simulink model "task3_simulation"  (R2025b)
settings: Solver=FixedStepAuto  StartTime=0.0  StopTime=45.4159  RelTol=1e-3
undefined symbols (not defined in the file): d, DiscIntNeverNeededParam, is_real_robot, k_theta, k_x, k_y, q_init, r, Ts, X, Y
libraries: robotlib x6, sharedtransform x1
settings Model: Creator=dallaliber  LastModifiedBy=ilia
settings OptimizationCC: DefaultParameterBehavior=Inlined  EnhancedBackFolding=on  PassReuseOutputArgsAs=Individual arguments  ZeroExternalMemoryAtStartup=off  ZeroInternalMemoryAtStartup=off  MaxStackSize=64  OptimizeBlockOrder=speed  DifferentSizesBufferReuse=on  OptimizationCustomize=off  EfficientTunableParamExpr=on
settings DebuggingCC: ParameterTunabilityLossMsg=error
settings HardwareCC: ProdBitPerPointer=32.0  ProdBitPerSizeT=32.0  ProdBitPerPtrDiffT=32.0  ProdLargestAtomicFloat=None  ProdIntDivRoundTo=Undefined  ProdEndianess=Unspecified  ProdWordSize=32.0  ProdHWDeviceType=Generic->Unspecified (assume 32-bit Generic)
settings SFSimCC: MATLABDynamicMemAlloc=off
settings RTWCC: SystemTargetFile=ert.tlc  HardwareBoard=Robot Operating System (ROS)  TLCOptions="-aInlineSetEventsForThisBaseRateFcn=TLC_FALSE -aSuppressMultiTaskScheduler=TLC_FALSE  -aRateBasedStepFcn=0"  TemplateMakefile=ert_default_tmf  Toolchain=Catkin  TargetLang=C++  Description=Embedded Coder
settings CodeAppCC: ForceParamTrailComments=on  IgnoreCustomStorageClasses=off  OperatorAnnotations=on  SimulinkDataObjDesc=on  SFDataObjDesc=on  InsertBlockDesc=on
settings ERTTargetCC: DynamicArrayContainerType=coder::array

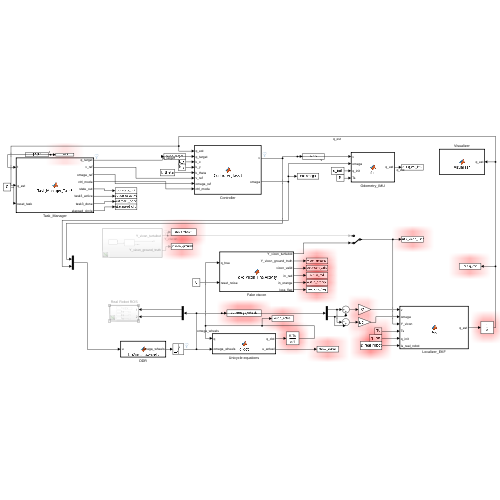
[thumbnail: Simulink's stored preview of the top-level diagram]
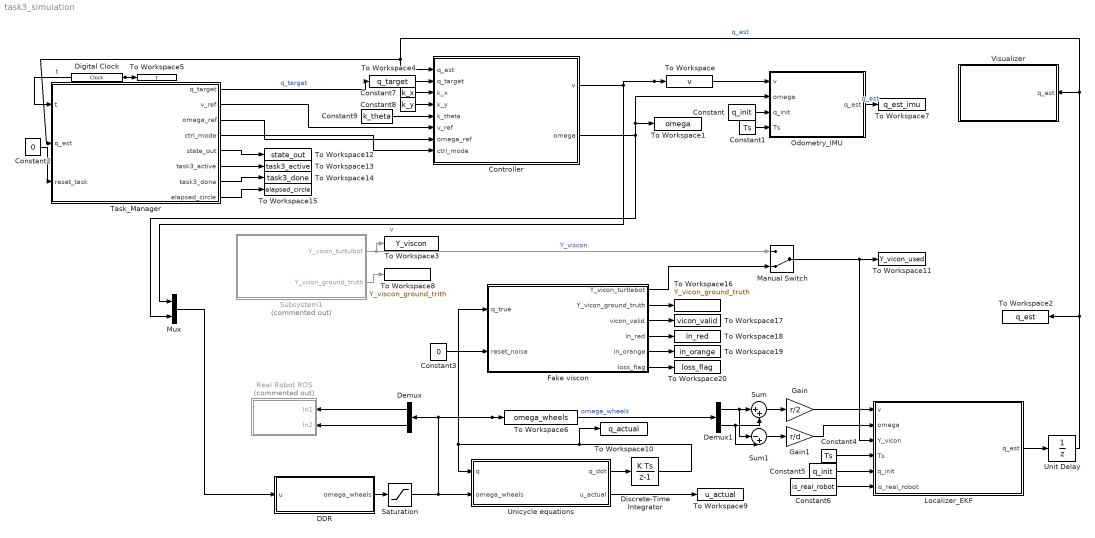
== system task3_simulation ==
  Constant : Constant  Value=q_init  SampleTime=Ts
  Constant1 : Constant  Value=Ts  SampleTime=Ts
  Constant2 : Constant  Value=0
  Constant3 : Constant  Value=0
  Constant4 : Constant  Value=Ts
  Constant5 : Constant  Value=q_init
  Constant6 : Constant  Value=is_real_robot
  Constant7 : Constant  Value=k_x  SampleTime=Ts
  Constant8 : Constant  Value=k_y  SampleTime=Ts
  Constant9 : Constant  Value=k_theta  SampleTime=Ts
  Controller : MATLAB Function  TreatAsAtomicUnit=on
  DDR : MATLAB Function  TreatAsAtomicUnit=on
  Demux : Demux  Outputs=2
  Demux1 : Demux  Outputs=2
  Digital Clock : DigitalClock  SampleTime=Ts
  Discrete-Time Integrator : DiscreteIntegrator  InitialCondition=q_init  SampleTime=Ts  ICPrevOutput=DiscIntNeverNeededParam  ICPrevScaledInput=DiscIntNeverNeededParam
  Fake viscon : MATLAB Function  TreatAsAtomicUnit=on
  Gain : Gain  Gain=r/2
  Gain1 : Gain  Gain=r/d
  Localizer_EKF : MATLAB Function  TreatAsAtomicUnit=on
  Manual Switch : ManualSwitch  CurrentSetting=0
  Mux : Mux  Inputs=2
  Odometry_IMU : MATLAB Function  TreatAsAtomicUnit=on
  Real Robot ROS : Subsystem  Commented=on
  Saturation : Saturate  UpperLimit=10  LowerLimit=-10
  Subsystem1 : Subsystem  Commented=on
  Sum : Sum  Inputs=|++
  Sum1 : Sum  Inputs=|-+
  Task_Manager : MATLAB Function  TreatAsAtomicUnit=on
  To Workspace : ToWorkspace  VariableName=v  SampleTime=Ts
  To Workspace1 : ToWorkspace  VariableName=omega  SampleTime=Ts
  To Workspace10 : ToWorkspace  VariableName=q_actual  SampleTime=Ts
  To Workspace11 : ToWorkspace  VariableName=Y_vicon_used  SampleTime=Ts
  To Workspace12 : ToWorkspace  VariableName=state_out  SampleTime=Ts
  To Workspace13 : ToWorkspace  VariableName=task3_active  SampleTime=Ts
  To Workspace14 : ToWorkspace  VariableName=task3_done  SampleTime=Ts
  To Workspace15 : ToWorkspace  VariableName=elapsed_circle  SampleTime=Ts
  To Workspace16 : ToWorkspace  VariableName=Y_vicon_ground_truth  SampleTime=Ts
  To Workspace17 : ToWorkspace  VariableName=vicon_valid  SampleTime=Ts
  To Workspace18 : ToWorkspace  VariableName=in_red  SampleTime=Ts
  To Workspace19 : ToWorkspace  VariableName=in_orange  SampleTime=Ts
  To Workspace2 : ToWorkspace  VariableName=q_est  SampleTime=Ts
  To Workspace20 : ToWorkspace  VariableName=loss_flag  SampleTime=Ts
  To Workspace3 : ToWorkspace  VariableName=Y_viscon  SampleTime=Ts
  To Workspace4 : ToWorkspace  VariableName=q_target  SampleTime=Ts
  To Workspace5 : ToWorkspace  VariableName=t  SampleTime=Ts
  To Workspace6 : ToWorkspace  VariableName=omega_wheels  SampleTime=Ts
  To Workspace7 : ToWorkspace  VariableName=q_est_imu  SampleTime=Ts
  To Workspace8 : ToWorkspace  VariableName=Y_viscon_ground_trith  SampleTime=Ts
  To Workspace9 : ToWorkspace  VariableName=u_actual  SampleTime=Ts
  Unicycle equations : MATLAB Function  TreatAsAtomicUnit=on
  Unit Delay : UnitDelay  InitialCondition=q_init  SampleTime=Ts  HasFrameUpgradeWarning=on
  Visualizer : MATLAB Function  TreatAsAtomicUnit=on
  wires:
  Controller/1(v) -> Odometry_IMU/1(v), To Workspace/1, Mux/1  "v"
  Constant/1 -> Odometry_IMU/3(q_init)
  Constant1/1 -> Odometry_IMU/4(Ts)
  Odometry_IMU/1(q_est) -> To Workspace7/1  "q_est"
  Saturation/1 -> Demux/1, To Workspace6/1, Demux1/1, Unicycle equations/2(omega_wheels)  "omega_wheels"
  DDR/1(omega_wheels) -> Saturation/1
  Demux/1 -> Real Robot ROS/1(In1)
  Mux/1 -> DDR/1(u)
  Digital Clock/1 -> To Workspace5/1, Task_Manager/1(t)  "t"
  Unit Delay/1 -> Controller/1(q_est), Task_Manager/2(q_est), Visualizer/1(q_est), To Workspace2/1  "q_est"
  Subsystem1/1(Y_vicon_turtulbot) -> To Workspace3/1, Manual Switch/1  "Y_viscon"
  Task_Manager/1(q_target) -> Controller/2(q_target), To Workspace4/1  "q_target"
  Constant7/1 -> Controller/3(k_x)
  Constant8/1 -> Controller/4(k_y)
  Subsystem1/2(Y_vicon_ground_truth) -> To Workspace8/1
  Constant9/1 -> Controller/5(k_theta)
  Controller/2(omega) -> To Workspace1/1, Odometry_IMU/2(omega), Mux/2
  Unicycle equations/1(q_dot) -> Discrete-Time Integrator/1
  Discrete-Time Integrator/1 -> To Workspace10/1, Unicycle equations/1(q), Fake viscon/1(q_true)
  Unicycle equations/2(u_actual) -> To Workspace9/1
  Fake viscon/1(Y_vicon_turtlebot) -> Manual Switch/2
  Constant4/1 -> Localizer_EKF/4(Ts)
  Constant6/1 -> Localizer_EKF/6(is_real_robot)
  Constant5/1 -> Localizer_EKF/5(q_init)
  Localizer_EKF/1(q_est) -> Unit Delay/1
  Demux/2 -> Real Robot ROS/2(In2)
  Demux1/1 -> Sum1/1, Sum/1
  Demux1/2 -> Sum/2, Sum1/2
  Sum/1 -> Gain/1
  Gain/1 -> Localizer_EKF/1(v)
  Sum1/1 -> Gain1/1
  Gain1/1 -> Localizer_EKF/2(omega)
  Manual Switch/1 -> To Workspace11/1, Localizer_EKF/3(Y_vicon)
  Constant2/1 -> Task_Manager/3(reset_task)
  Task_Manager/2(v_ref) -> Controller/6(v_ref)
  Constant3/1 -> Fake viscon/2(reset_noise)
  Fake viscon/2(Y_vicon_ground_truth) -> To Workspace16/1
  Fake viscon/3(vicon_valid) -> To Workspace17/1
  Fake viscon/4(in_red) -> To Workspace18/1
  Fake viscon/5(in_orange) -> To Workspace19/1
  Fake viscon/6(loss_flag) -> To Workspace20/1
  Task_Manager/3(omega_ref) -> Controller/7(omega_ref)
  Task_Manager/4(ctrl_mode) -> Controller/8(ctrl_mode)
  Task_Manager/5(state_out) -> To Workspace12/1
  Task_Manager/6(task3_active) -> To Workspace13/1
  Task_Manager/7(task3_done) -> To Workspace14/1
  Task_Manager/8(elapsed_circle) -> To Workspace15/1

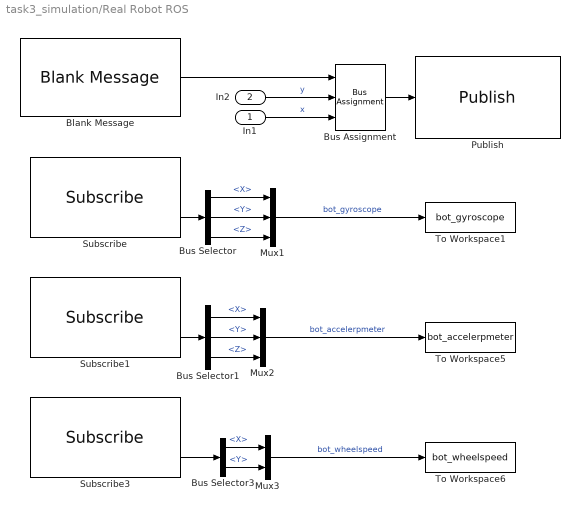
== system task3_simulation/Real Robot ROS ==
  In1 : Inport
  In2 : Inport  Port=2
  Blank Message : robotlib/Blank Message  messageClass=Message  entityType=geometry_msgs/Vector3  messageType=geometry_msgs/Vector3  SampleTime=0.04  legacyBusStruct=off
  Bus Assignment : BusAssignment  AssignedSignals=X,Y
  Bus Selector : BusSelector  OutputSignals=X,Y,Z
  Bus Selector1 : BusSelector  OutputSignals=X,Y,Z
  Bus Selector3 : BusSelector  OutputSignals=X,Y
  Mux1 : Mux  Inputs=3
  Mux2 : Mux  Inputs=3
  Mux3 : Mux  Inputs=2
  Publish : robotlib/Publish  topicSource=Select from ROS network  topic=/turtlebot_09/cmd_wheels  messageType=geometry_msgs/Vector3  legacyBusStruct=off  messageQueueLength=1
  Subscribe : robotlib/Subscribe  topicSource=Select from ROS network  topic=/turtlebot_09/gyroscope  messageType=geometry_msgs/Vector3  SampleTime=0.04  legacyBusStruct=off  messageQueueLength=1
  Subscribe1 : robotlib/Subscribe  topicSource=Select from ROS network  topic=/turtlebot_09/accelerometer  messageType=geometry_msgs/Vector3  SampleTime=0.04  legacyBusStruct=off  messageQueueLength=1
  Subscribe3 : robotlib/Subscribe  topicSource=Select from ROS network  topic=/turtlebot_09/wheelSpeeds  messageType=geometry_msgs/Vector3  SampleTime=0.04  legacyBusStruct=off  messageQueueLength=1
  To Workspace1 : ToWorkspace  VariableName=bot_gyroscope  SaveFormat=Timeseries  SampleTime=Ts
  To Workspace5 : ToWorkspace  VariableName=bot_accelerpmeter  SaveFormat=Timeseries  SampleTime=Ts
  To Workspace6 : ToWorkspace  VariableName=bot_wheelspeed  SaveFormat=Timeseries  SampleTime=Ts
  wires:
  Subscribe1/2 -> Bus Selector1/1
  Bus Selector1/1 -> Mux2/1  "<X>"
  Mux2/1 -> To Workspace5/1  "bot_accelerpmeter"
  Bus Assignment/1 -> Publish/1
  Subscribe/2 -> Bus Selector/1
  Bus Selector/2 -> Mux1/2  "<Y>"
  Bus Selector/1 -> Mux1/1  "<X>"
  Bus Selector3/1 -> Mux3/1  "<X>"
  Bus Selector3/2 -> Mux3/2  "<Y>"
  Bus Selector1/3 -> Mux2/3  "<Z>"
  Bus Selector1/2 -> Mux2/2  "<Y>"
  Mux3/1 -> To Workspace6/1  "bot_wheelspeed"
  Mux1/1 -> To Workspace1/1  "bot_gyroscope"
  Subscribe3/2 -> Bus Selector3/1
  Blank Message/1 -> Bus Assignment/1
  Bus Selector/3 -> Mux1/3  "<Z>"
  In1/1 -> Bus Assignment/3  "x"
  In2/1 -> Bus Assignment/2  "y"

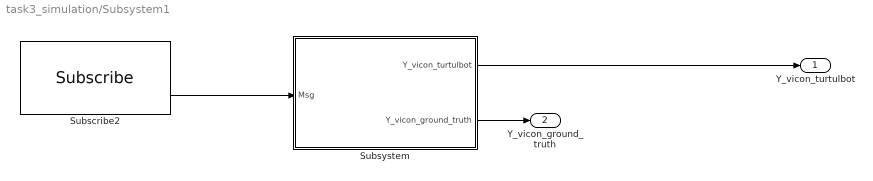
== system task3_simulation/Subsystem1 ==
  Subscribe2 : robotlib/Subscribe  topicSource=Select from ROS network  topic=/turtlebot_09/odom  messageType=nav_msgs/Odometry  SampleTime=Ts  legacyBusStruct=off  messageQueueLength=1
      settings: LibrarySourceBlock=roslib/ROS/Subscribe
  Subsystem : Subsystem
  Y_vicon_turtulbot : Outport
  Y_vicon_ground_truth : Outport  Port=2
  wires:
  Subscribe2/2 -> Subsystem/1(Msg)
  Subsystem/2(Y_vicon_ground_truth) -> Y_vicon_ground_truth/1
  Subsystem/1(Y_vicon_turtulbot) -> Y_vicon_turtulbot/1

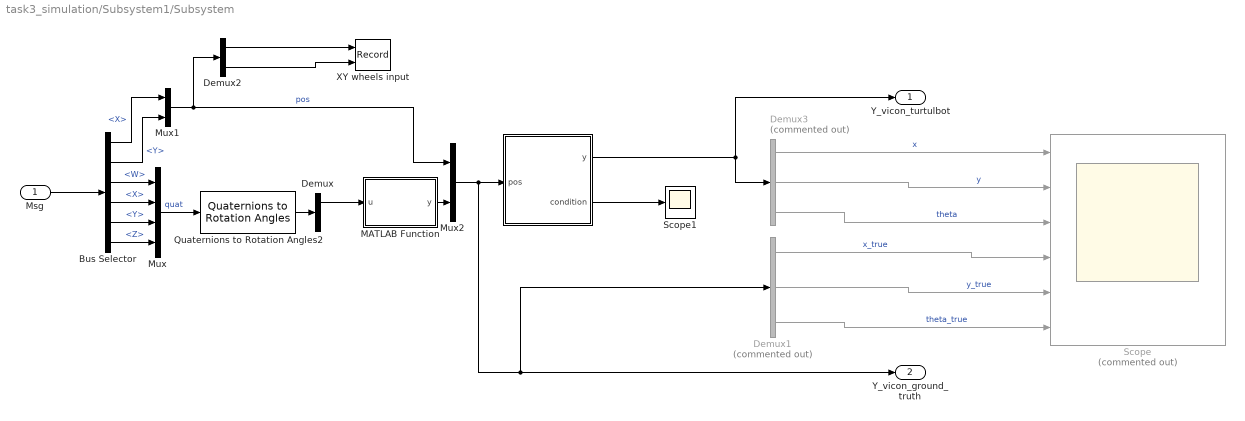
== system task3_simulation/Subsystem1/Subsystem ==
  Msg : Inport
  " " : MATLAB Function  TreatAsAtomicUnit=on
  Bus Selector : BusSelector  OutputSignals=Pose.Pose.Position.X,Pose.Pose.Position.Y,Pose.Pose.Orientation.W,Pose.Pose.Orientation.X,Pose.Pose.Orientation.Y,Pose.Pose.Orientation.Z
  Demux : Demux  Outputs=3
  Demux1 : Demux  Commented=on  Outputs=3
  Demux2 : Demux  Outputs=2
  Demux3 : Demux  Commented=on  Outputs=3
  MATLAB Function : MATLAB Function  TreatAsAtomicUnit=on
  Mux : Mux
  Mux1 : Mux  Inputs=2
  Mux2 : Mux  Inputs=2
  Quaternions to Rotation Angles2 : sharedtransform/Quaternions to Rotation Angles  rotationOrder=ZYX  aMode=aMode
  Scope : Scope  Commented=on  NumInputPorts=6
      settings: ActiveDisplayYMinimum=-0.22169  ActiveDisplayYMaximum=1.9952
  Scope1 : Scope
  XY wheels input : Record  NumPorts=2.0  FileSettingsInternal="{\"entries\":[{\"content\":{\"excelSettings\":{\"content\":{},\"type\":\"Streamout.ExcelSettings\"},\"parquetSettings\":{\"content\":{},\"type\":\"Streamout.ParquetSettings\"}},\"type\":\"Streamout.FileSettingStorage\",\"uuid\":\"\"}],\"packageUris\":[\"http:\\/\\/schema.mathworks.com\\/mf0\\/streamout_blocks\\/R2020a\"],\"version\":\"1.0\"}"  FrameSettings=[0, 0]  Layout=[1 1]  SignalsInternal="{\"entries\":[{\"content\":{\"signals\":[{\"content\":{\"blockPath\":[],\"dimensions\":[1],\"domain\":\"\",\"lineColor\":\"#7e2f8e\",\"lineWidth\":2,\"port\":1,\"signalID\":1,\"signalName\":\"Demux2:1\"},\"type\":\"RecordBlkView.Signal\",\"uuid\":\"\"},{\"content\":{\"blockPath\":[],\"dimensions\":[1],\"domain\":\"\",\"lineColor\":\"#77ac30\",\"lineWidth\":2,\"port\":2,\"signalID\":2,\"signalName\":\"Demux2:2\"},\"type\":\"RecordBlkView.Signal\",\"uuid\":\"\"}]},\"type\":\"RecordBlkView.InputSignals\",\"uuid\":\"\"}],\"packageUris\":[\"http:\\/\\/schema.mathworks.com\\/mf0\\/streamout_blocks\\/R2020a\"],\"version\":\"1.0\"}"  VisualizationBindings="{\"xyplotplugin\":{\"info\":[{\"series\":[],\"subplotID\":1}]}}"  CompatibilityTag=XY
  Y_vicon_turtulbot : Outport
  Y_vicon_ground_truth : Outport  Port=2
  wires:
  Msg/1 -> Bus Selector/1
  Mux2/1 -> Demux1/1, Y_vicon_ground_truth/1, " "/1(pos)
  Bus Selector/3 -> Mux/1  "<W>"
  Mux/1 -> Quaternions to Rotation Angles2/1  "quat"
  Bus Selector/2 -> Mux1/2  "<Y>"
  Demux3/1 -> Scope/1  "x"
  Bus Selector/6 -> Mux/4  "<Z>"
  Bus Selector/1 -> Mux1/1  "<X>"
  " "/1(y) -> Y_vicon_turtulbot/1, Demux3/1
  Demux1/2 -> Scope/5  "y_true"
  Bus Selector/4 -> Mux/2  "<X>"
  Bus Selector/5 -> Mux/3  "<Y>"
  Demux1/3 -> Scope/6  "theta_true"
  " "/2(condition) -> Scope1/1
  Demux3/3 -> Scope/3  "theta"
  Demux3/2 -> Scope/2  "y"
  Demux1/1 -> Scope/4  "x_true"
  MATLAB Function/1(y) -> Mux2/2
  Mux1/1 -> Demux2/1, Mux2/1  "pos"
  Quaternions to Rotation Angles2/1 -> Demux/1
  Demux/1 -> MATLAB Function/1(u)
  Demux2/1 -> XY wheels input/1
  Demux2/2 -> XY wheels input/2

== matlab function task3_simulation/DDR ==
  data: u input; omega_wheels output; r parameter; d parameter
function omega_wheels = kin2omegawheels(u, r, d)
omega_l = u(1)/r-d/(2*r)*u(2);
omega_r = u(1)/r+d/(2*r)*u(2);
omega_wheels = [omega_l;omega_r];

== matlab function task3_simulation/Unicycle equations ==
  data: q input; omega_wheels input; q_dot output; r parameter; d parameter; u_actual output
function [q_dot, u_actual] = q_dot(q, omega_wheels, r, d)
u_actual = [r/2, r/2;-r/d, r/d]*omega_wheels;
theta = q(3);
q_dot = [[cos(theta), 0];[sin(theta), 0];[0,1]]*u_actual;

== matlab function task3_simulation/Task_Manager ==
  data: t input; q_est input; q_target output; reset_task input; v_ref output; omega_ref output; ctrl_mode output; state_out output; task3_active output; task3_done output; elapsed_circle output
function [q_target, v_ref, omega_ref, ctrl_mode, state_out, task3_active, task3_done, elapsed_circle] = Task_Manager(t, q_est, reset_task)
%#codegen
% Task 3 manager:
% State 1: move from Task 2 end to Task 3 circular start
% State 2: circular trajectory tracking
% State 3: stop / hold final pose

persistent state t_circle0 q_hold

if isempty(state) || reset_task > 0.5
    state = 1;
    t_circle0 = 0.0;
    q_hold = zeros(3,1);
end

%% ============================================================
% Task 3 geometry
% ============================================================

% Task 3 starting point: [x8, y4]
x_start = 1.45;
y_start = -0.30;

% Cube / circle center
xc = 2.00;
yc = 0.00;

dx0 = x_start - xc;
dy0 = y_start - yc;

R_circle = sqrt(dx0^2 + dy0^2);

% Counter-clockwise circle
circle_dir = 1.0;

% Circle angular speed
omega_circle_abs = 0.30;      % [rad/s]

% One and a half turns
N_turns = 1.5;
T_circle = 2*pi*N_turns/omega_circle_abs;

% Initial angular coordinate on circle
alpha0 = atan2(dy0, dx0);

% Tangent heading at the circle start
theta_start = wrapToPiLocal(alpha0 + circle_dir*pi/2);

q_start = zeros(3,1);
q_start(1) = x_start;
q_start(2) = y_start;
q_start(3) = theta_start;

%% ============================================================
% Switching thresholds
% ============================================================
% These numbers are chosen to avoid two bad cases:
% 1) starting the circle too early with bad heading;
% 2) stopping forever at the start point.

pos_thr_start   = 0.050;     % [m]
theta_thr_start = 0.05;      % [rad], about 20 deg

%% ============================================================
% Default outputs
% ============================================================

q_target = zeros(3,1);
q_target(1) = q_start(1);
q_target(2) = q_start(2);
q_target(3) = q_start(3);

v_ref = 0.0;
omega_ref = 0.0;
ctrl_mode = 1.0;
elapsed_circle = 0.0;

%% ============================================================
% State 1: go to circular start
% ============================================================

if state == 1

    q_target(1) = q_start(1);
    q_target(2) = q_start(2);
    q_target(3) = q_start(3);

    v_ref = 0.0;
    omega_ref = 0.0;
    ctrl_mode = 1.0;

    ex = q_start(1) - q_est(1);
    ey = q_start(2) - q_est(2);
    eth = wrapToPiLocal(q_start(3) - q_est(3));

    pos_err = sqrt(ex^2 + ey^2);
    theta_err = abs(eth);

    normal_switch = (pos_err < pos_thr_start) && (theta_err < theta_thr_start);

    if normal_switch
        state = 2;
        t_circle0 = t;
        elapsed_circle = 0.0;
    end
end

%% ============================================================
% State 2: circular tracking
% ============================================================

if state == 2

    elapsed_circle = t - t_circle0;

    if elapsed_circle < 0.0
        elapsed_circle = 0.0;
    end

    if elapsed_circle > T_circle
        elapsed_circle = T_circle;
    end

    alpha = alpha0 + circle_dir*omega_circle_abs*elapsed_circle;

    xd = xc + R_circle*cos(alpha);
    yd = yc + R_circle*sin(alpha);
    thd = wrapToPiLocal(alpha + circle_dir*pi/2);

    q_target(1) = xd;
    q_target(2) = yd;
    q_target(3) = thd;

    v_ref = R_circle*omega_circle_abs;
    omega_ref = circle_dir*omega_circle_abs;

    ctrl_mode = 2.0;

    if (t - t_circle0) >= T_circle
        q_hold(1) = q_target(1);
        q_hold(2) = q_target(2);
        q_hold(3) = q_target(3);
        state = 3;
    end
end

%% ============================================================
% State 3: stop / hold final pose
% ============================================================

if state == 3

    q_target(1) = q_hold(1);
    q_target(2) = q_hold(2);
    q_target(3) = q_hold(3);

    v_ref = 0.0;
    omega_ref = 0.0;
    ctrl_mode = 3.0;
    elapsed_circle = T_circle;
end

%% ============================================================
% Outputs
% ============================================================

state_out = state;
task3_active = double(state == 2);
task3_done = double(state == 3);

end

function a = wrapToPiLocal(a)
a = atan2(sin(a), cos(a));
end

== matlab function task3_simulation/Controller ==
  data: q_est input; v output; q_target input; k_x input; k_y input; k_theta input; omega output; v_ref input; omega_ref input; ctrl_mode input
function [v, omega] = Controller(q_est, q_target, k_x, k_y, k_theta, v_ref, omega_ref, ctrl_mode)
%#codegen
% Task 3 controller:
% ctrl_mode = 1: regulation to Task 3 start point
% ctrl_mode = 2: circular trajectory tracking
% ctrl_mode = 3: stop

theta = q_est(3);

dx = q_target(1) - q_est(1);
dy = q_target(2) - q_est(2);
dtheta = wrapToPiLocal(q_target(3) - q_est(3));

%% Safety limits
v_lim = 0.22;
omega_lim = 0.60;

%% ============================================================
% Mode 2: circular trajectory tracking
% ============================================================

if ctrl_mode == 2

    % Error expressed in robot frame
    e1 =  cos(theta)*dx + sin(theta)*dy;
    e2 = -sin(theta)*dx + cos(theta)*dy;
    e3 = dtheta;

    if abs(e3) < 1e-4
        sinc_e3 = 1.0;
    else
        sinc_e3 = sin(e3)/e3;
    end

    % Tuned circular tracking gains
    k1 = 0.70;
    k2 = 2.30;
    k3 = 0.7;

    v = v_ref*cos(e3) + k1*e1;

    omega = omega_ref ...
          + k2*v_ref*sinc_e3*e2 ...
          + k3*e3;

%% ============================================================
% Mode 1: regulation to the circular start point
% ============================================================

elseif ctrl_mode == 1

    rho = sqrt(dx^2 + dy^2);
    angle_to_goal = atan2(dy, dx);
    alpha = wrapToPiLocal(angle_to_goal - theta);

    % Regulation gains
    k_rho   = 0.55;
    k_alpha = 1.20;
    k_final = 0.95;

    % Important:
    % rho_switch must be smaller than pos_thr_start in Task_Manager.
    % Task_Manager pos_thr_start = 0.060
    rho_switch = 0.005;

    if rho > rho_switch

        v = k_rho*rho*cos(alpha);

        % If the robot is badly oriented toward the point, avoid cutting.
        if abs(alpha) > 1.2
            v = 0.0;
        elseif abs(alpha) > 0.6
            v = 0.4*v;
        end

        omega = k_alpha*alpha;

    else

        % Close to the start point:
        % stop translation and align heading with the circle tangent.
        v = 0.0;
        omega = k_final*dtheta;

    end

%% ============================================================
% Mode 3: stop
% ============================================================

else

    v = 0.0;
    omega = 0.0;

end

%% Saturation
v = satLocal(v, -v_lim, v_lim);
omega = satLocal(omega, -omega_lim, omega_lim);

end

function y = satLocal(u, umin, umax)
y = min(max(u, umin), umax);
end

function a = wrapToPiLocal(a)
a = atan2(sin(a), cos(a));
end

== matlab function task3_simulation/Odometry_IMU ==
  data: v input; q_est output; omega input; q_init input; Ts input
function q_est = fcn(v, omega, q_init, Ts)
    % Persistent variables hold their value between function calls
    persistent q_prev;
    
    if isempty(q_prev)
        q_prev = q_init;
    end
    
    % Dead-reckoning equations
    theta_new = q_prev(3) + omega * Ts;
    
    % Ensure angle is wrapped between -pi and pi
    theta_new = wrapToPi(theta_new);
    
    x_new = q_prev(1) + v * cos(theta_new) * Ts;
    y_new = q_prev(2) + v * sin(theta_new) * Ts;
    
    q_est = [x_new; y_new; theta_new];
    q_prev = q_est;
end

== matlab function task3_simulation/Fake viscon ==
  data: q_true input; Y_vicon_turtlebot output; reset_noise input; Y_vicon_ground_truth output; vicon_valid output; in_red output; in_orange output; loss_flag output
function [Y_vicon_turtlebot, Y_vicon_ground_truth, ...
          vicon_valid, in_red, in_orange, loss_flag] = Fake_Vicon_FinalActivity(q_true, reset_noise)
%#codegen
% Fake Vicon block consistent with the final activity rules.
%
% Red area: Gaussian noise, sigma_e = 0.02.
% Orange area: measurement loss with p_loss = 0.9.
% Missing measurement is returned as [0;0;0].
% Ground truth is always available only for analysis.

persistent seed

if isempty(seed) || reset_noise > 0.5
    seed = 123456789.0;
end

%% =========================
%  Map coordinates
%  =========================
x5  = -0.60;
x6  =  0.20;
x7  =  1.00;
x11 =  2.90;

y1 = -1.50;
y6 =  0.10;
y8 =  1.50;

%% =========================
%  Parameters
%  =========================
sigma_e = 0.02;     % Gaussian noise standard deviation
p_loss  = 0.90;     % loss probability in orange area

%% =========================
%  True pose
%  =========================
x = q_true(1);
y = q_true(2);
theta = wrapToPiLocal(q_true(3));

Y_vicon_ground_truth = [x; y; theta];

%% =========================
%  Region checks
%  =========================
in_red = double((x >= x5) && (x <= x6) && (y >= y1) && (y <= y6));

in_orange = double((x >= x7) && (x <= x11) && (y >= y1) && (y <= y8));

%% =========================
%  Default output: clean measurement
%  =========================
Y_vicon_turtlebot = Y_vicon_ground_truth;
vicon_valid = 1.0;
loss_flag = 0.0;

%% =========================
%  Apply final-activity measurement rules
%  =========================

if in_orange > 0.5
    % In orange area: measurement is lost with probability p_loss.
    [u, seed] = uniformLCG(seed);

    if u < p_loss
        Y_vicon_turtlebot = [0.0; 0.0; 0.0];
        vicon_valid = 0.0;
        loss_flag = 1.0;
    else
        % Available measurement in orange area.
        % Keep it clean unless you explicitly want extra noise.
        Y_vicon_turtlebot = Y_vicon_ground_truth;
        vicon_valid = 1.0;
        loss_flag = 0.0;
    end

elseif in_red > 0.5
    % In red area: Gaussian corrupted measurement.
    [n1, seed] = gaussianLCG(seed);
    [n2, seed] = gaussianLCG(seed);
    [n3, seed] = gaussianLCG(seed);

    Y_vicon_turtlebot = Y_vicon_ground_truth + sigma_e * [n1; n2; n3];
    Y_vicon_turtlebot(3) = wrapToPiLocal(Y_vicon_turtlebot(3));

    vicon_valid = 1.0;
    loss_flag = 0.0;

else
    % Normal area: clean motion capture.
    Y_vicon_turtlebot = Y_vicon_ground_truth;
    vicon_valid = 1.0;
    loss_flag = 0.0;
end

end

%% ==========================================================
%  Local helper functions
%  ==========================================================

function [u, seed] = uniformLCG(seed)
% Deterministic pseudo-random generator.
% This avoids relying on rand/randn inside Simulink code generation.

a = 1664525.0;
c = 1013904223.0;
m = 4294967296.0;   % 2^32

seed = mod(a*seed + c, m);

% Avoid exactly 0 or 1.
u = (seed + 1.0) / (m + 2.0);
end

function [z, seed] = gaussianLCG(seed)
% Gaussian random number using Box-Muller transform.

[u1, seed] = uniformLCG(seed);
[u2, seed] = uniformLCG(seed);

if u1 < 1e-12
    u1 = 1e-12;
end

z = sqrt(-2.0*log(u1)) * cos(2.0*pi*u2);
end

function a = wrapToPiLocal(a)
a = atan2(sin(a), cos(a));
end

== matlab function task3_simulation/Visualizer ==
  data: q_est input
function visualizer(q_est)
    coder.extrinsic('draw_robot');
    draw_robot(q_est(1), q_est(2));
end

== matlab function task3_simulation/Subsystem1/Subsystem/  ==
  data: y output; pos input; condition output
function [y, condition] = check(pos)

x1 = -2.9; y1 = -1.5;
x2 = -1.6; y2 = -1.1;
x3 = -1.5; y3 = -0.7;
x4 = -1.4; y4 = -0.3;
x5 = -0.6; y5 =  0.1;
x6 =  0.2; y6 =  1.5;
x7 =  1.0;
x8 =  1.1;
x9 =  2.9;

P_loss = 0.9;


if ((pos(1) >= x5) && (pos(1) <= x6)) && ((pos(2) >= y1) && (pos(2) <= y5))
    % add noise
    y = pos + 0.02*randn(3,1);
    condition = 1;
elseif ((pos(1) >= x7) && (pos(1) <= x9)) && ((pos(2) >= y1) && (pos(2) <= y6))
    % measurement loss
    if rand > P_loss
        y = pos;
    else
        y = 0*pos;
    end
    condition = 2;
else
    y = pos;
    condition = 0;
end

== matlab function task3_simulation/Localizer_EKF ==
  data: v input; omega input; Y_vicon input; Ts input; q_est output; q_init input; is_real_robot input
function q_est = fcn(v, omega, Y_vicon, Ts, q_init, is_real_robot)
% EKF-based localizer for TurtleBot Task 2
%
% Prediction:
%   Unicycle model using odometric inputs v and omega.
%
% Update:
%   Vicon pose measurement when available.
%
% In the red area, the Vicon measurement covariance is increased,
% so the EKF trusts the odometric prediction more than the noisy Vicon.

persistent q_hat P Q initialized

%% ============================================================
% 1. Initialization
% ============================================================

if isempty(initialized)

    if is_real_robot == 1
        % Real robot mode:
        % Wait until a valid Vicon measurement is available.
        if all(Y_vicon == 0)
            q_est = q_init;
            return;
        else
            q_hat = Y_vicon;
            q_hat(3) = localWrapToPi(q_hat(3));
            initialized = true;
        end

    else
        % Simulation mode:
        % Start directly from the selected initial condition.
        q_hat = q_init;
        q_hat(3) = localWrapToPi(q_hat(3));
        initialized = true;
    end

    % Initial covariance
    P = eye(3) * 0.1;

    % Process noise covariance:
    % uncertainty of the odometric/unicycle prediction.
    Q = diag([1e-4, 1e-4, 5e-4]);
end

%% ============================================================
% 2. Prediction step
% ============================================================

theta = q_hat(3);

% Unicycle model prediction
q_pred = q_hat + [v*cos(theta); ...
                  v*sin(theta); ...
                  omega] * Ts;

q_pred(3) = localWrapToPi(q_pred(3));

% Jacobian of the prediction model with respect to the state
F = [1, 0, -v*sin(theta)*Ts;
     0, 1,  v*cos(theta)*Ts;
     0, 0,  1];

% Covariance prediction
P = F * P * F' + Q;

%% ============================================================
% 3. Measurement validity and red-area detection
% ============================================================

% Missing Vicon measurement is represented as [0; 0; 0]
is_lost = all(Y_vicon == 0);

% Red noisy Vicon area:
% x5 <= x <= x6 and y1 <= y <= y6
in_red = (q_pred(1) >= -0.60 && q_pred(1) <= 0.20 && ...
          q_pred(2) >= -1.50 && q_pred(2) <= 0.10);

%% ============================================================
% 4. Measurement covariance
% ============================================================

if in_red
    % In the red area, Vicon is noisy.
    % Therefore, the filter trusts the Vicon correction less.
    R = diag([0.7, 0.7, 0.9]);
else
    % Outside the red area, Vicon is assumed to be reliable.
    R = diag([1e-5, 1e-5, 5e-5]);
end

%% ============================================================
% 5. Update step
% ============================================================

if is_lost
    % If Vicon is not available, use only the prediction.
    q_est = q_pred;

else
    % Measurement model:
    % Vicon directly measures [x; y; theta]
    H = eye(3);

    % Kalman gain
    K = (P * H') / (H * P * H' + R);

    % Innovation
    innovation = Y_vicon - q_pred;
    innovation(3) = localWrapToPi(innovation(3));

    % State correction
    q_est = q_pred + K * innovation;
    q_est(3) = localWrapToPi(q_est(3));

    % Covariance correction
    P = (eye(3) - K * H) * P;
end

% Store estimate for next sample
q_hat = q_est;

end

%% ============================================================
% Local angle wrapping function
% ============================================================

function a = localWrapToPi(a)
a = atan2(sin(a), cos(a));
end

== matlab function task3_simulation/Subsystem1/Subsystem/MATLAB Function ==
  data: u input; y output
function y = manual_unwrap(u)
    % این تابع به صورت دستی عملیات Unwrap را برای سیگنال‌های ورودی انجام می‌دهد.
    
    persistent prev_u cumulative_offset
    
    % مقداردهی اولیه در اولین گام اجرای شبیه‌سازی
    if isnan(u)
        u = 0;
    end
    if isempty(prev_u)
        prev_u = u;
        cumulative_offset = zeros(size(u));
    end
    
    % محاسبه اختلاف زاویه فعلی با قبلی
    diff = u - prev_u;
    
    % شناسایی پرش‌های بزرگتر از 180 درجه (pi رادیان)
    for i = 1:length(u)
        if diff(i) > pi
            cumulative_offset(i) = cumulative_offset(i) - 2*pi;
        elseif diff(i) < -pi
            cumulative_offset(i) = cumulative_offset(i) + 2*pi;
        end
    end
    
    % اعمال آفست تجمعی به ورودی فعلی
    y = u + cumulative_offset;
    
    % ذخیره مقدار فعلی برای استفاده در گام بعدی
    prev_u = u;

end
